simulink library "linkage_bushing_6DOF_lib"  (R2025a)
settings: Solver=VariableStepAuto  StartTime=0.0  StopTime=10.0  RelTol=1e-3
undefined symbols (not defined in the file): Connection, d_axialX, d_axialY, d_axialZ, d_torsX, d_torsY, d_torsZ, f_axialX_dam, f_axialX_spr, f_axialY_dam, f_axialY_spr, f_axialZ_dam, f_axialZ_spr, hp_joint, k_axialX, k_axialY, k_axialZ, k_torsX, k_torsY, k_torsZ, Linear, m_spr, m_sprX, m_sprZ, m_torsY, m_torsZ, m_torX, q_spr, q_sprX, q_sprZ, rhs_y, Table, v_axialX, v_axialY, v_axialZ, Visual, w_torsY, w_torsZ, w_torX, X, x_axialX, x_axialY, x_axialZ, Y, Z
libraries: sm_lib x22, Suspension_Utilities x7, $bdroot x3, bushing_forces_lib x2, linkage_bushing_5DOF_lib x1
(part 1 of 2)
Description:
  | Component of Simscape Vehicle Templates Library
  | 
  | Copyright 2018-2026 The MathWorks, Inc.
settings Model: Creator=smiller  LastModifiedBy=smiller
settings OptimizationCC: ReuseModelBlockBuffer=off
settings ModelReferenceCC: EnableRefExpFcnMdlSchedulingChecks=on
settings RTWCC: GPUComputeCapability=3.5

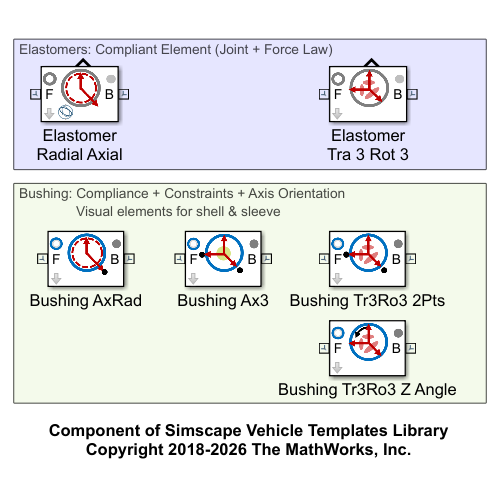
[thumbnail: Simulink's stored preview of the top-level diagram]
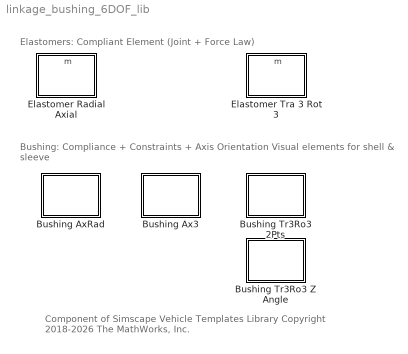
== system linkage_bushing_6DOF_lib ==
  note: Component of Simscape Vehicle Templates Library
      | Copyright 2018-2026 The MathWorks, Inc.
  note: Elastomers: Compliant Element (Joint + Force Law)
  note: Bushing: Compliance + Constraints + Axis Orientation
      |                Visual elements for shell & sleeve
  Bushing Ax3 : Subsystem  VariantControl=Bushing_Ax3  mask(Bushing with Independent Axial Compliance on 3-Axes (6-DOF)){checkbox_setTargets=on, leftOrRight=rhs_y, hp_j=hp_joint, hp_z=Connection.sAxialOrientationZ.Value, hp_x=Connection.sAxialOrientationX.Value, AxisAttachment=Connection.AxisAttachment.class.Value, sprx=Connection.SpringX, spry=Connection.SpringY, sprz=Connection.SpringZ, damx=Connection.DamperX, damy=Connection.DamperY, damz=Connection.DamperZ, shell_or=Visual.hp.rad*2, shell_len=Visual.hp.rad*2, shell_clr=Visual.BushingShell.clr, shell_opc=Visual.part.opc, sleeve_clr=Visual.Bushing.clr, sleeve_opc=Visual.part.opc}
      mask prompts: checkbox_setTargets "Set position targets to 0"; leftOrRight "Left (1) or Right (-1)"; hp_j "Joint HP [x  y z] (m)"; hp_z "Bushing Z-Axis Point [x y z] (m)"; hp_x "Bushing X-Axis Point [x y z] (m)"; AxisAttachment "Bushing Axes Attachment (string)"; sprx "Spring X Parameters (struct)"; spry "Spring Y Parameters (struct)"; sprz "Spring Z Parameters (struct)"; damx "Damper X Parameters (struct)"; damy "Damper Y Parameters (struct)"; damz "Damper Z Parameters (struct)"; shell_or "Shell Outer Radius (m)"; shell_len "Shell Length (m)"; shell_clr "Shell Color [R G B]"; shell_opc "Shell Opacity (0-1)"; sleeve_clr "Sleeve Color [R G B]"; sleeve_opc "Sleeve Opacity (0-1)"
      mask help: Models bushing compliance with independent force laws for x, y, and z directions. Select force laws that model compliance as linear or nonlinear.
      mask init:
      | curblk = gcb;
      | 
      | set_param([curblk '/Elastomer'],...
      |     'popup_force_law_spr_axiX', sprx.Law.Value,...
      |     'popup_force_law_spr_axiY', spry.Law.Value,...
      |     'popup_force_law_spr_axiZ', sprz.Law.Value,...
      |     'popup_force_law_dam_axiX', damx.Law.Value,...
      |     'popup_force_law_dam_axiY', damy.Law.Value,...
      |     'popup_force_law_dam_axiZ', damz.Law.Value...
      |     );
      | 
      | if(strcmp(AxisAttachment,'Inner'))
      |    set_param([curblk '/Inner'],'LabelModeActiveChoice','Fixed');
      |    set_param([curblk '/Outer'],'LabelModeActiveChoice','Gimbal');
      | elseif(strcmp(AxisAttachment,'Outer'))
      |    set_param([curblk '/Inner'],'LabelModeActiveChoice','Revolute');
      |    set_param([curblk '/Outer'],'LabelModeActiveChoice','Universal');
      | end
      | 
      | leftOrRight_vec = [1 leftOrRight 1];
      mask TypeOptions checkbox_setTargets: Inner/checkbox_setTargets | Outer/checkbox_setTargets | Elastomer/checkbox_setTargets
      mask TypeOptions hp_j: Elastomer/hp_j
      mask DialogControl cont_vis Prompt: Visualization
      mask Display: image('sm_car_bushing_tr3_perpaxial.png');
  Bushing AxRad : Subsystem  VariantControl=Bushing_AxRad  mask(Bushing with Radial and Axial Compliance, 6 DOF){checkbox_setTargets=on, leftOrRight=rhs_y, hp_j=hp_joint, hp_z=Connection.sAxialOrientationZ.Value, sprRad=Connection.RadialSpring, damRad=Connection.RadialDamper, sprAxi=Connection.AxialSpring, damAxi=Connection.AxialSpring, shell_or=Visual.hp.rad*2, shell_len=Visual.hp.rad*2, shell_clr=Visual.BushingShell.clr, shell_opc=Visual.part.opc, sleeve_clr=Visual.Bushing.clr, sleeve_opc=Visual.part.opc}
      mask prompts: checkbox_setTargets "Set position targets to 0"; leftOrRight "Left (1) or Right (-1)"; hp_j "Joint HP [x  y z] (m)"; hp_z "Bushing Z-Axis Point [x y z] (m)"; sprRad "Radial Spring Parameters (struct)"; damRad "Radial Darmper Parameters (struct)"; sprAxi "Axial Spring Parameters (struct)"; damAxi "Axial Damper Parameters (struct)"; shell_or "Shell Outer Radius (m)"; shell_len "Shell Length (m)"; shell_clr "Shell Color [R G B]"; shell_opc "Shell Opacity (0-1)"; sleeve_clr "Sleeve Color [R G B]"; sleeve_opc "Sleeve Opacity (0-1)"
      mask help: Models compliance with independent radial and axial force laws. Specify orientation of axial axis by defining the location of the bushing and the location of a point along that axis.
      mask init:
      | curblk = gcb;
      | set_param([curblk '/Elastomer'],...
      |     'popup_force_law_dam_rad', damRad.Law.Value,...
      |     'popup_force_law_spr_axi', sprAxi.Law.Value,...
      |     'popup_force_law_dam_axi', damAxi.Law.Value...
      |     );
      | set_param([curblk '/Elastomer'],...
      |     'popup_force_law_spr_rad', sprAxi.Law.Value);
      | 
      | leftOrRight_vec = [1 leftOrRight 1];
      mask TypeOptions checkbox_setTargets: Elastomer/checkbox_setTargets
      mask TypeOptions hp_j: Elastomer/hp_j
      mask DialogControl cont_vis Prompt: Visualization
      mask Display: image('sm_car_bushing_axrad_6dof.png');
  Bushing Tr3Ro3 2Pts : Subsystem  VariantControl=Bushing_Tr3Ro3  mask(Bushing with Axial and Torsional Compliance, Orient Two Points){checkbox_setTargets=on, leftOrRight=rhs_y, hp_j=hp_joint, hp_z=Connection.sAxialOrientationZ.Value, hp_x=Connection.sAxialOrientationX.Value, sprx=Connection.SpringX, spry=Connection.SpringY, sprz=Connection.SpringZ, damx=Connection.DamperX, damy=Connection.DamperY, damz=Connection.DamperZ, sprqx=Connection.SpringqX, sprqy=Connection.SpringqY, sprqz=Connection.SpringqZ, damqx=Connection.DamperqX, damqy=Connection.DamperqY, damqz=Connection.DamperqZ, shell_or=Visual.hp.rad*2, shell_len=Visual.hp.rad*2, shell_clr=Visual.BushingShell.clr, shell_opc=Visual.part.opc, sleeve_clr=Visual.Bushing.clr, sleeve_opc=Visual.part.opc}
      mask prompts: checkbox_setTargets "Set position targets to 0"; leftOrRight "Left (1) or Right (-1)"; hp_j "HP Joint [xyz] (m)"; hp_z "Bushing Z-Axis Point [x y z] (m)"; hp_x "Bushing X-Axis Point [x y z] (m)"; sprx "Spring X Parameters (struct)"; spry "Spring Y Parameters (struct)"; sprz "Spring Z Parameters (struct)"; damx "Damper X Parameters (struct)"; damy "Damper Y Parameters (struct)"; damz "Damper Z Parameters (struct)"; sprqx "Spring X Parameters (struct)"; sprqy "Spring Y Parameters (struct)"; sprqz "Spring Z Parameters (struct)"; damqx "Damper X Parameters (struct)"; damqy "Damper Y Parameters (struct)"; damqz "Damper Z Parameters (struct)"; shell_or "Shell Outer Radius (m)"; shell_len "Shell Length (m)"; shell_clr "Shell Color [R G B]"; shell_opc "Shell Opacity (0-1)"; sleeve_clr "Sleeve Color [R G B]"; sleeve_opc "Sleeve Opacity (0-1)"
      mask help: Models bushing compliance with independent force laws for translational and rotational stiffness and damping. The forces are parameterized along/about each local axis. Select force laws that model compliance as a linear coefficient or a lookup table. Orientation of z- and x- axes are defined by two points in 3D space.
      mask init:
      | curblk = gcb;
      | 
      | set_param([curblk '/Elastomer'],...
      |     'popup_force_law_spr_axiX', sprx.Law.Value,...
      |     'popup_force_law_spr_axiY', spry.Law.Value,...
      |     'popup_force_law_spr_axiZ', sprz.Law.Value,...
      |     'popup_force_law_dam_axiX', damx.Law.Value,...
      |     'popup_force_law_dam_axiY', damy.Law.Value,...
      |     'popup_force_law_dam_axiZ', damz.Law.Value,...
      |     'popup_force_law_spr_torX', sprqx.Law.Value,...
      |     'popup_force_law_spr_torY', sprqy.Law.Value,...
      |     'popup_force_law_spr_torZ', sprqz.Law.Value,...
      |     'popup_force_law_dam_torX', damqx.Law.Value,...
      |     'popup_force_law_dam_torY', damqy.Law.Value,...
      |     'popup_force_law_dam_torZ', damqz.Law.Value...
      |     );
      | 
      | leftOrRight_vec = [1 leftOrRight 1];
      mask TypeOptions checkbox_setTargets: Elastomer/checkbox_setTargets
      mask DialogControl cont_trans Prompt: Translational
      mask DialogControl cont_rot Prompt: Rotational
      mask DialogControl cont_vis Prompt: Visualization
      mask Display: image('sm_car_bushing_tr3ro3_2pts.png');
  Bushing Tr3Ro3 Z Angle : Subsystem  VariantControl=Bushing_Tr3Ro3  mask(Bushing with Axial and Torsional Compliance, Orient Z-Axis Rotation){checkbox_setTargets=on, leftOrRight=rhs_y, qOriZ=Connection.qOriZ.Value, sprx=Connection.SpringX, spry=Connection.SpringY, sprz=Connection.SpringZ, damx=Connection.DamperX, damy=Connection.DamperY, damz=Connection.DamperZ, sprqx=Connection.SpringqX, sprqy=Connection.SpringqY, sprqz=Connection.SpringqZ, damqx=Connection.DamperqX, damqy=Connection.DamperqY, damqz=Connection.DamperqZ, shell_or=Visual.hp.rad*2, shell_len=Visual.hp.rad*2, shell_clr=Visual.BushingShell.clr, shell_opc=Visual.part.opc, sleeve_clr=Visual.Bushing.clr, sleeve_opc=Visual.part.opc}
      mask prompts: checkbox_setTargets "Set position targets to 0"; leftOrRight "Left (1) or Right (-1)"; qOriZ "Z-Axis Rotation (deg)"; sprx "Spring X Parameters (struct)"; spry "Spring Y Parameters (struct)"; sprz "Spring Z Parameters (struct)"; damx "Damper X Parameters (struct)"; damy "Damper Y Parameters (struct)"; damz "Damper Z Parameters (struct)"; sprqx "Spring X Parameters (struct)"; sprqy "Spring Y Parameters (struct)"; sprqz "Spring Z Parameters (struct)"; damqx "Damper X Parameters (struct)"; damqy "Damper Y Parameters (struct)"; damqz "Damper Z Parameters (struct)"; shell_or "Shell Outer Radius (m)"; shell_len "Shell Length (m)"; shell_clr "Shell Color [R G B]"; shell_opc "Shell Opacity (0-1)"; sleeve_clr "Sleeve Color [R G B]"; sleeve_opc "Sleeve Opacity (0-1)"
      mask help: Models bushing compliance with independent force laws for translational and rotational stiffness and damping. The forces are parameterized along/about each local axis. Select force laws that model compliance as a linear coefficient or a lookup table. Orientation of x- and y-axis are defined a rotation angle about the z-axis.
      mask init: same as linkage_bushing_6DOF_lib/Bushing Tr3Ro3 2Pts
      mask TypeOptions checkbox_setTargets: Elastomer/checkbox_setTargets
      mask DialogControl cont_trans Prompt: Translational
      mask DialogControl cont_rot Prompt: Rotational
      mask DialogControl cont_vis Prompt: Visualization
      mask Display: image('sm_car_bushing_tr3ro3_zangle.png')
  Elastomer Radial Axial : Subsystem  mask(Elastomer with Radial and Axial Compliance (6-DOF)){checkbox_setTargets=off, popup_force_law_spr_rad=Linear, k_radial=20, x_radial=[-4, -3, -2, -1, 0, 1, 2, 3, 4], f_radial_spr=[-4, -3, -2, -1, 0, 1, 2, 3, 4]*10, k1_radial_max=3.0139e+03, b1_radial_max=11471, x_radial_max=[-3 -1.5 1.5 3]*1e-3, f_radial_max=[-10 -4 4 10]*655.5098, popup_force_law_dam_rad=Linear, d_radial=20, v_radial=[-4, -3, -2, -1, 0, 1, 2, 3, 4], f_radial_dam=[-4, -3, -2, -1, 0, 1, 2, 3, 4]*10, popup_force_law_spr_axi=Linear, k_axial=20, x_axial=[-4, -3, -2, -1, 0, 1, 2, 3, 4], f_axial_spr=[-4, -3, -2, -1, 0, 1, 2, 3, 4]*10, popup_force_law_dam_axi=Linear, d_axial=20, v_axial=[-4, -3, -2, -1, 0, 1, 2, 3, 4], f_axial_dam=[-4, -3, -2, -1, 0, 1, 2, 3, 4]*10, shell_or=Visual.hp.rad*2, elastomer_ir=Visual.hp.rad, shell_len=Visual.hp.rad*4, elastomer_clr=Visual.Bushing.clr, elastomer_opc=Visual.part.opc}
      mask prompts: checkbox_setTargets "Set position targets to 0"; popup_force_law_spr_rad "Spring Force Law"; k_radial "Spring Coefficient (N/mm)"; x_radial "Spring Deflection [min max] (mm)"; f_radial_spr "Spring Force [min max] (N)"; k1_radial_max "Maxwell k1"; b1_radial_max "Maxwell b1"; x_radial_max "Maxwell Displacement [min max] (mm)"; f_radial_max "Maxwell Force [min max] (N)"; popup_force_law_dam_rad "Damper Force Law"; d_radial "Damper Coefficient (N/(m/s))"; v_radial "Damper Velocity [min max] (m/s)"; f_radial_dam "Damper Force [min max] (N)"; popup_force_law_spr_axi "Spring Force Law"; k_axial "Spring Coefficient (N/mm)"; x_axial "Spring Displacement [min max] (mm)"; f_axial_spr "Spring Force [min max] (N)"; popup_force_law_dam_axi "Damper Force Law"; d_axial "Damper Coefficient (N/(m/s))"; v_axial "Damper Velocity [min max] (m/s)"; f_axial_dam "Damper Force [min max] (N)"; shell_or "Shell Outer Radius (m)"; elastomer_ir "Elastomer Inner Radius (m)"; shell_len "Shell Length (m)"; elastomer_clr "Elastomer Color [R G B]"; elastomer_opc "Elastomer Opacity [R G B]"
      mask help: Models elastomer compliance with independent force laws for radial (x-y plane) and axial (z-axis) directions. Select force laws that model compliance as linear, nonlinear, or nonlinear with hysteresis. All 6 degrees of freedom are provided within this block to make the overall model more efficient.
      mask init:
      | curblk = gcb;
      | if(checkbox_setTargets)
      |     set_param([curblk '/Elastomer Joint'],...
      |         'PxPositionTargetSpecify','on',...
      |         'PyPositionTargetSpecify','on',...
      |         'PzPositionTargetSpecify','on',...
      |         'RxPositionTargetSpecify','on',...
      |         'RyPositionTargetSpecify','on',...
      |         'RzPositionTargetSpecify','on'...
      |         );
      | else
      |     set_param([curblk '/Elastomer Joint'],...
      |         'PxPositionTargetSpecify','off',...
      |         'PyPositionTargetSpecify','off',...
      |         'PzPositionTargetSpecify','off',...
      |         'RxPositionTargetSpecify','off',...
      |         'RyPositionTargetSpecify','off',...
      |         'RzPositionTargetSpecify','off'...
      |         );
      | end
      settings: PortSchema="{\"entries\":[{\"content\":{\"sides\":[{\"content\":{\"connectorIds\":[\"LConn1\"]},\"type\":\"ConnectorPlacement.EquallySpacedRectSide\",\"uuid\":\"540bb151-3239-4a9d-82ba-b7afa97281a8\"},{\"content\":{\"connectorIds\":[\"RConn1\"],\"side\":\"RIGHT\"},\"type\":\"ConnectorPlacement.EquallySpacedRectSide\",\"uuid\":\"0af2999e-e304-4113-9c38-08ac5dd2068d\"},{\"content\":{\"connectorIds\":[\"Out1\"],\"side\":\"TOP\"},\"type\":\"ConnectorPlacement.EquallySpacedRectSide\",\"uuid\":\"c7e19545-6bd3-4656-b994-719fb436eca6\"}]},\"type\":\"ConnectorPlacement.EquallySpacedConnector\",\"uuid\":\"c532a1d4-44be-42d7-8101-c903e69d0a9b\"}],\"packageUris\":[\"http://schema.mathworks.com/mf0/Connector/R2020b\"],\"version\":\"1.0\"}"
      mask TypeOptions popup_force_law_spr_rad: Force Law/popup_force_law_spr_rad
      mask Callback popup_force_law_spr_rad:
      | maskObj = Simulink.Mask.get(gcb); % Get the mask object of the current block
      | krad_h  = maskObj.getParameter('k_radial'); % Get the parameter to hide
      | 
      | xrad_h  = maskObj.getParameter('x_radial'); % Get the parameter to hide
      | fSrad_h = maskObj.getParameter('f_radial_spr'); % Get the parameter to hide
      | k1rad_h  = maskObj.getParameter('k1_radial_max'); % Get the parameter to hide
      | b1rad_h  = maskObj.getParameter('b1_radial_max'); % Get the parameter to hide
      | xmrad_h  = maskObj.getParameter('x_radial_max'); % Get the parameter to hide
      | fmrad_h  = maskObj.getParameter('f_radial_max'); % Get the parameter to hide
      | 
      | % Check the value of ControlParam
      | frcLawSpr = get_param(gcb, 'popup_force_law_spr_rad');
      | 
      | krad_h.Visible  = 'off';
      | xrad_h.Visible  = 'off';
      | fSrad_h.Visible = 'off';
      | k1rad_h.Visible  = 'off';
      | b1rad_h.Visible  = 'off';
      | xmrad_h.Visible  = 'off';
      | fmrad_h.Visible  = 'off';
      | 
      | if strcmp(frcLawSpr, 'Linear')
      |     krad_h.Visible  = 'on';
      | elseif strcmp(frcLawSpr, 'Table')
      |     xrad_h.Visible  = 'on';
      |     fSrad_h.Visible = 'on';
      | elseif strcmp(frcLawSpr, 'Maxwell_SLS')
      |     k1rad_h.Visible  = 'on';
      |     b1rad_h.Visible = 'on';
      |     xmrad_h.Visible = 'on';
      |     fmrad_h.Visible = 'on';
      | end
      mask TypeOptions k_radial: Force Law/k_radial
      mask TypeOptions x_radial: Force Law/x_radial
      mask TypeOptions f_radial_spr: Force Law/f_radial_spr
      mask TypeOptions k1_radial_max: Force Law/k1_radial_max
      mask TypeOptions b1_radial_max: Force Law/b1_radial_max
      mask TypeOptions x_radial_max: Force Law/x_radial_max
      mask TypeOptions f_radial_max: Force Law/f_radial_max
      mask TypeOptions popup_force_law_dam_rad: Force Law/popup_force_law_dam_rad
      mask Callback popup_force_law_dam_rad:
      | maskObj = Simulink.Mask.get(gcb); % Get the mask object of the current block
      | drad_h  = maskObj.getParameter('d_radial'); % Get the parameter to hide
      | 
      | vrad_h  = maskObj.getParameter('v_radial'); % Get the parameter to hide
      | fDrad_h = maskObj.getParameter('f_radial_dam'); % Get the parameter to hide
      | 
      | % Check the value of ControlParam
      | frcLawDam = get_param(gcb, 'popup_force_law_dam_rad');
      | 
      | drad_h.Visible  = 'off';
      | vrad_h.Visible  = 'off';
      | fDrad_h.Visible = 'off';
      | 
      | if strcmp(frcLawDam, 'Linear')
      |     drad_h.Visible  = 'on';
      | elseif strcmp(frcLawDam, 'Table')
      |     vrad_h.Visible  = 'on';
      |     fDrad_h.Visible = 'on';
      | end
      mask TypeOptions d_radial: Force Law/d_radial
      mask TypeOptions v_radial: Force Law/v_radial
      mask TypeOptions f_radial_dam: Force Law/f_radial_dam
      mask TypeOptions popup_force_law_spr_axi: Force Law/popup_force_law_spr_axi
      mask Callback popup_force_law_spr_axi:
      | maskObj = Simulink.Mask.get(gcb); % Get the mask object of the current block
      | kaxi_h  = maskObj.getParameter('k_axial'); % Get the parameter to hide
      | 
      | xaxi_h  = maskObj.getParameter('x_axial'); % Get the parameter to hide
      | fSaxi_h  = maskObj.getParameter('f_axial_spr'); % Get the parameter to hide
      | 
      | % Check the value of ControlParam
      | controlParamValue = get_param(gcb, 'popup_force_law_spr_axi');
      | 
      | kaxi_h.Visible  = 'off';
      | xaxi_h.Visible  = 'off';
      | fSaxi_h.Visible  = 'off';
      | 
      | if strcmp(controlParamValue, 'Linear')
      |     kaxi_h.Visible  = 'on';
      | else
      |     xaxi_h.Visible  = 'on';
      |     fSaxi_h.Visible  = 'on';
      | end
      mask TypeOptions k_axial: Force Law/k_axial
      mask TypeOptions x_axial: Force Law/x_axial
      mask TypeOptions f_axial_spr: Force Law/f_axial_spr
      mask TypeOptions popup_force_law_dam_axi: Force Law/popup_force_law_dam_axi
      mask Callback popup_force_law_dam_axi:
      | maskObj = Simulink.Mask.get(gcb); % Get the mask object of the current block
      | daxi_h  = maskObj.getParameter('d_axial'); % Get the parameter to hide
      | 
      | vaxi_h  = maskObj.getParameter('v_axial'); % Get the parameter to hide
      | fDaxi_h  = maskObj.getParameter('f_axial_dam'); % Get the parameter to hide
      | 
      | % Check the value of ControlParam
      | controlParamValue = get_param(gcb, 'popup_force_law_dam_axi');
      | 
      | daxi_h.Visible  = 'off';
      | vaxi_h.Visible  = 'off';
      | fDaxi_h.Visible  = 'off';
      | 
      | if strcmp(controlParamValue, 'Linear')
      |     daxi_h.Visible  = 'on';
      | else
      |     vaxi_h.Visible  = 'on';
      |     fDaxi_h.Visible  = 'on';
      | end
      mask TypeOptions d_axial: Force Law/d_axial
      mask TypeOptions v_axial: Force Law/v_axial
      mask TypeOptions f_axial_dam: Force Law/f_axial_dam
      mask DialogControl cont_radial Prompt: Radial
      mask DialogControl cont_axial Prompt: Axial
      mask DialogControl cont_vis Prompt: Visualization
      mask Display: image('sm_car_elastomer_axrad_6dof.png');
  Elastomer Tra 3 Rot 3 : Subsystem  mask(Elastomer with Axial  and Torsional Compliance){checkbox_setTargets=off, popup_force_law_spr_axiX=Table, k_axialX=k_axialX, x_axialX=x_axialX, f_axialX_spr=f_axialX_spr, popup_force_law_dam_axiX=Linear, d_axialX=d_axialX, v_axialX=v_axialX, f_axialX_dam=f_axialX_dam, popup_force_law_spr_axiY=Linear, k_axialY=k_axialY, x_axialY=x_axialY, f_axialY_spr=f_axialY_spr, popup_force_law_dam_axiY=Linear, d_axialY=d_axialY, v_axialY=v_axialY, f_axialY_dam=f_axialY_dam, popup_force_law_spr_axiZ=Linear, k_axialZ=k_axialZ, x_axialZ=x_axialZ, f_axialZ_spr=f_axialZ_spr, popup_force_law_dam_axiZ=Linear, d_axialZ=d_axialZ, v_axialZ=v_axialZ, f_axialZ_dam=f_axialZ_dam, popup_force_law_spr_torX=Linear, k_torsX=k_torsX, q_sprX=q_sprX, m_sprX=m_sprX, popup_force_law_dam_torX=Linear, d_torsX=d_torsX, w_torsX=w_torX, m_torsX=m_torX, popup_force_law_spr_torY=Table, k_torsY=k_torsY, q_sprY=q_spr, m_sprY=m_spr, popup_force_law_dam_torY=Table, d_torsY=d_torsY, w_torsY=w_torsY, m_torsY=m_torsY, popup_force_law_spr_torZ=Linear, k_torsZ=k_torsZ, q_sprZ=q_sprZ, m_sprZ=m_sprZ, popup_force_law_dam_torZ=Linear, d_torsZ=d_torsZ, w_torsZ=w_torsZ, m_torsZ=m_torsZ, shell_or=Visual.hp.rad*2, elastomer_ir=Visual.hp.rad, shell_len=Visual.hp.rad*2, elastomer_clr=Visual.Bushing.clr, elastomer_opc=Visual.part.opc, elastomer_axis_clr=Visual.BushingXAxis.clr}
      mask prompts: checkbox_setTargets "Set position targets to 0"; popup_force_law_spr_axiX "Spring Force Law"; k_axialX "Spring Coefficient (N/mm)"; x_axialX "Spring Displacement [min max] (mm)"; f_axialX_spr "Spring Force [min max] (N)"; popup_force_law_dam_axiX "Damper Force Law"; d_axialX "Damper Coefficient (N/(m/s))"; v_axialX "Damper Velocity [min max] (m/s)"; f_axialX_dam "Damper Force [min max] (N)"; popup_force_law_spr_axiY "Spring Force Law"; k_axialY "Spring Coefficient (N/mm)"; x_axialY "Spring Displacement [min max] (mm)"; f_axialY_spr "Spring Force [min max] (N)"; popup_force_law_dam_axiY "Damper Force Law"; d_axialY "Damper Coefficient (N/(m/s))"; v_axialY "Damper Velocity [min max] (m/s)"; f_axialY_dam "Damper Force [min max] (N)"; popup_force_law_spr_axiZ "Spring Force Law"; k_axialZ "Spring Coefficient (N/mm)"; x_axialZ "Spring Displacement [min max] (mm)"; f_axialZ_spr "Spring Force [min max] (N)"; popup_force_law_dam_axiZ "Damper Force Law"; d_axialZ "Damper Coefficient (N/(m/s))"; v_axialZ "Damper Velocity [min max] (m/s)"; f_axialZ_dam "Damper Force [min max] (N)"; popup_force_law_spr_torX "Spring Force Law"; k_torsX "Spring Coefficient  (N*m/deg)"; q_sprX "Spring Displacement [min max] (deg)"; m_sprX "Spring Torque [min max] (N*m)"; popup_force_law_dam_torX "Damper Force Law"; d_torsX "Damper Coefficient (N*m/(deg/s))"; w_torsX "Damper Velocity [min max] (deg/s)"; m_torsX "Damper Torque [min max] (N*m)"; popup_force_law_spr_torY "Spring Force Law"; k_torsY "Spring Coefficient (N*m/deg)"; q_sprY "Spring Displacement [min max] (deg)"; m_sprY "Spring Torque [min max] (N*m)"; popup_force_law_dam_torY "Damper Force Law"; d_torsY "Damper Coefficient (N*m/(deg/s))"; w_torsY "Damper Velocity [min max] (deg/s)"; m_torsY "Damper Torque [min max] (N*m)"; popup_force_law_spr_torZ "Spring Force Law"; k_torsZ "Spring Coefficient (N*m/deg)"; q_sprZ "Spring Displacement [min max] (deg)"; m_sprZ "Spring Torque [min max] (N*m)"; popup_force_law_dam_torZ "Damper Force Law"; d_torsZ "Damper Coefficient (N*m/(deg/s))"; w_torsZ "Damper Velocity [min max] (deg/s)"; m_torsZ "Damper Torque [min max] (N*m)"; shell_or "Shell Outer Radius (m)"; elastomer_ir "Elastomer Inner Radius (m)"; shell_len "Shell Length (m)"; elastomer_clr "Elastomer Color [R G B]"; elastomer_opc "Elastomer Opacity [R G B]"; elastomer_axis_clr "Elastomer Axis Color [R G B]"
      mask help: Models elastomer compliance with independent force laws for translational and rotational stiffness and damping. The forces are parameterized along/about each local axis. Select force laws that model compliance as a linear coefficient or a lookup table.
      mask init: same as linkage_bushing_6DOF_lib/Elastomer Radial Axial
      settings: PortSchema="{\"entries\":[{\"content\":{\"sides\":[{\"content\":{\"connectorIds\":[\"LConn1\"]},\"type\":\"ConnectorPlacement.EquallySpacedRectSide\",\"uuid\":\"540bb151-3239-4a9d-82ba-b7afa97281a8\"},{\"content\":{\"connectorIds\":[\"RConn1\"],\"side\":\"RIGHT\"},\"type\":\"ConnectorPlacement.EquallySpacedRectSide\",\"uuid\":\"0af2999e-e304-4113-9c38-08ac5dd2068d\"},{\"content\":{\"connectorIds\":[\"Out1\"],\"side\":\"TOP\"},\"type\":\"ConnectorPlacement.EquallySpacedRectSide\",\"uuid\":\"c7e19545-6bd3-4656-b994-719fb436eca6\"}]},\"type\":\"ConnectorPlacement.EquallySpacedConnector\",\"uuid\":\"c532a1d4-44be-42d7-8101-c903e69d0a9b\"}],\"packageUris\":[\"http://schema.mathworks.com/mf0/Connector/R2020b\"],\"version\":\"1.0\"}"
      mask TypeOptions popup_force_law_spr_axiX: Force Law/popup_force_law_spr_axiX
      mask Callback popup_force_law_spr_axiX:
      | maskObj = Simulink.Mask.get(gcb); % Get the mask object of the current block
      | kaxiX_h  = maskObj.getParameter('k_axialX'); % Get the parameter to hide
      | 
      | xaxiX_h  = maskObj.getParameter('x_axialX'); % Get the parameter to hide
      | fSaxiX_h  = maskObj.getParameter('f_axialX_spr'); % Get the parameter to hide
      | 
      | % Check the value of ControlParam
      | controlParamValue = get_param(gcb, 'popup_force_law_spr_axiX');
      | 
      | kaxiX_h.Visible  = 'off';
      | xaxiX_h.Visible  = 'off';
      | fSaxiX_h.Visible  = 'off';
      | 
      | if strcmp(controlParamValue, 'Linear')
      |     kaxiX_h.Visible  = 'on';
      | else
      |     xaxiX_h.Visible  = 'on';
      |     fSaxiX_h.Visible  = 'on';
      | end
      mask TypeOptions k_axialX: Force Law/k_axialX
      mask TypeOptions x_axialX: Force Law/x_axialX
      mask TypeOptions f_axialX_spr: Force Law/f_axialX_spr
      mask TypeOptions popup_force_law_dam_axiX: Force Law/popup_force_law_dam_axiX
      mask Callback popup_force_law_dam_axiX:
      | maskObj = Simulink.Mask.get(gcb); % Get the mask object of the current block
      | daxiX_h  = maskObj.getParameter('d_axialX'); % Get the parameter to hide
      | 
      | vaxiX_h  = maskObj.getParameter('v_axialX'); % Get the parameter to hide
      | fDaxiX_h  = maskObj.getParameter('f_axialX_dam'); % Get the parameter to hide
      | 
      | % Check the value of ControlParam
      | controlParamValue = get_param(gcb, 'popup_force_law_dam_axiX');
      | 
      | daxiX_h.Visible  = 'off';
      | vaxiX_h.Visible  = 'off';
      | fDaxiX_h.Visible  = 'off';
      | 
      | if strcmp(controlParamValue, 'Linear')
      |     daxiX_h.Visible  = 'on';
      | else
      |     vaxiX_h.Visible  = 'on';
      |     fDaxiX_h.Visible  = 'on';
      | end
      mask TypeOptions d_axialX: Force Law/d_axialX
      mask TypeOptions v_axialX: Force Law/v_axialX
      mask TypeOptions f_axialX_dam: Force Law/f_axialX_dam
      mask TypeOptions popup_force_law_spr_axiY: Force Law/popup_force_law_spr_axiY
      mask Callback popup_force_law_spr_axiY:
      | maskObj = Simulink.Mask.get(gcb); % Get the mask object of the current block
      | kaxiY_h  = maskObj.getParameter('k_axialY'); % Get the parameter to hide
      | 
      | xaxiY_h  = maskObj.getParameter('x_axialY'); % Get the parameter to hide
      | fSaxiY_h  = maskObj.getParameter('f_axialY_spr'); % Get the parameter to hide
      | 
      | % Check the value of ControlParam
      | controlParamValue = get_param(gcb, 'popup_force_law_spr_axiY');
      | 
      | kaxiY_h.Visible  = 'off';
      | xaxiY_h.Visible  = 'off';
      | fSaxiY_h.Visible  = 'off';
      | 
      | if strcmp(controlParamValue, 'Linear')
      |     kaxiY_h.Visible  = 'on';
      | else
      |     xaxiY_h.Visible  = 'on';
      |     fSaxiY_h.Visible  = 'on';
      | end
      mask TypeOptions k_axialY: Force Law/k_axialY
      mask TypeOptions x_axialY: Force Law/x_axialY
      mask TypeOptions f_axialY_spr: Force Law/f_axialY_spr
      mask TypeOptions popup_force_law_dam_axiY: Force Law/popup_force_law_dam_axiY
      mask Callback popup_force_law_dam_axiY:
      | maskObj = Simulink.Mask.get(gcb); % Get the mask object of the current block
      | daxiY_h  = maskObj.getParameter('d_axialY'); % Get the parameter to hide
      | 
      | vaxiY_h  = maskObj.getParameter('v_axialY'); % Get the parameter to hide
      | fDaxiY_h  = maskObj.getParameter('f_axialY_dam'); % Get the parameter to hide
      | 
      | % Check the value of ControlParam
      | controlParamValue = get_param(gcb, 'popup_force_law_dam_axiY');
      | 
      | daxiY_h.Visible  = 'off';
      | vaxiY_h.Visible  = 'off';
      | fDaxiY_h.Visible  = 'off';
      | 
      | if strcmp(controlParamValue, 'Linear')
      |     daxiY_h.Visible  = 'on';
      | else
      |     vaxiY_h.Visible  = 'on';
      |     fDaxiY_h.Visible  = 'on';
      | end
      mask TypeOptions d_axialY: Force Law/d_axialY
      mask TypeOptions v_axialY: Force Law/v_axialY
      mask TypeOptions f_axialY_dam: Force Law/f_axialY_dam
      mask TypeOptions popup_force_law_spr_axiZ: Force Law/popup_force_law_spr_axiZ
      mask Callback popup_force_law_spr_axiZ:
      | maskObj = Simulink.Mask.get(gcb); % Get the mask object of the current block
      | kaxiZ_h  = maskObj.getParameter('k_axialZ'); % Get the parameter to hide
      | 
      | xaxiZ_h  = maskObj.getParameter('x_axialZ'); % Get the parameter to hide
      | fSaxiZ_h  = maskObj.getParameter('f_axialZ_spr'); % Get the parameter to hide
      | 
      | % Check the value of ControlParam
      | controlParamValue = get_param(gcb, 'popup_force_law_spr_axiZ');
      | 
      | kaxiZ_h.Visible  = 'off';
      | xaxiZ_h.Visible  = 'off';
      | fSaxiZ_h.Visible  = 'off';
      | 
      | if strcmp(controlParamValue, 'Linear')
      |     kaxiZ_h.Visible  = 'on';
      | else
      |     xaxiZ_h.Visible  = 'on';
      |     fSaxiZ_h.Visible  = 'on';
      | end
      mask TypeOptions k_axialZ: Force Law/k_axialZ
      mask TypeOptions x_axialZ: Force Law/x_axialZ
      mask TypeOptions f_axialZ_spr: Force Law/f_axialZ_spr
      mask TypeOptions popup_force_law_dam_axiZ: Force Law/popup_force_law_dam_axiZ
      mask Callback popup_force_law_dam_axiZ:
      | maskObj = Simulink.Mask.get(gcb); % Get the mask object of the current block
      | daxiZ_h  = maskObj.getParameter('d_axialZ'); % Get the parameter to hide
      | 
      | vaxiZ_h  = maskObj.getParameter('v_axialZ'); % Get the parameter to hide
      | fDaxiZ_h  = maskObj.getParameter('f_axialZ_dam'); % Get the parameter to hide
      | 
      | % Check the value of ControlParam
      | controlParamValue = get_param(gcb, 'popup_force_law_dam_axiZ');
      | 
      | daxiZ_h.Visible  = 'off';
      | vaxiZ_h.Visible  = 'off';
      | fDaxiZ_h.Visible  = 'off';
      | 
      | if strcmp(controlParamValue, 'Linear')
      |     daxiZ_h.Visible  = 'on';
      | else
      |     vaxiZ_h.Visible  = 'on';
      |     fDaxiZ_h.Visible  = 'on';
      | end
      mask TypeOptions d_axialZ: Force Law/d_axialZ
      mask TypeOptions v_axialZ: Force Law/v_axialZ
      mask TypeOptions f_axialZ_dam: Force Law/f_axialZ_dam
      mask TypeOptions popup_force_law_spr_torX: Force Law/popup_force_law_spr_torX
      mask Callback popup_force_law_spr_torX:
      | maskObj = Simulink.Mask.get(gcb); % Get the mask object of the current block
      | ktorX_h  = maskObj.getParameter('k_torsX'); % Get the parameter to hide
      | 
      | qsprX_h  = maskObj.getParameter('q_sprX'); % Get the parameter to hide
      | msprX_h  = maskObj.getParameter('m_sprX'); % Get the parameter to hide
      | 
      | % Check the value of ControlParam
      | controlParamValue = get_param(gcb, 'popup_force_law_spr_torX');
      | 
      | ktorX_h.Visible  = 'off';
      | qsprX_h.Visible  = 'off';
      | msprX_h.Visible  = 'off';
      | 
      | if strcmp(controlParamValue, 'Linear')
      |     ktorX_h.Visible  = 'on';
      | elseif strcmp(controlParamValue, 'Table')
      |     qsprX_h.Visible  = 'on';
      |     msprX_h.Visible  = 'on';
      | end
      mask TypeOptions k_torsX: Force Law/k_torsX
      mask TypeOptions q_sprX: Force Law/q_sprX
      mask TypeOptions m_sprX: Force Law/m_sprX
      mask TypeOptions popup_force_law_dam_torX: Force Law/popup_force_law_dam_torX
      mask Callback popup_force_law_dam_torX:
      | maskObj = Simulink.Mask.get(gcb); % Get the mask object of the current block
      | dtorX_h  = maskObj.getParameter('d_torsX'); % Get the parameter to hide
      | 
      | wtorX_h  = maskObj.getParameter('w_torsX'); % Get the parameter to hide
      | mtorX_h  = maskObj.getParameter('m_torsX'); % Get the parameter to hide
      | 
      | % Check the value of ControlParam
      | controlParamValue = get_param(gcb, 'popup_force_law_dam_torX');
      | 
      | dtorX_h.Visible  = 'off';
      | wtorX_h.Visible  = 'off';
      | mtorX_h.Visible  = 'off';
      | 
      | if strcmp(controlParamValue, 'Linear')
      |     dtorX_h.Visible  = 'on';
      | else
      |     wtorX_h.Visible  = 'on';
      |     mtorX_h.Visible  = 'on';
      | end
      mask TypeOptions d_torsX: Force Law/d_torsX
      mask TypeOptions w_torsX: Force Law/w_torsX
      mask TypeOptions m_torsX: Force Law/m_torsX
      mask TypeOptions popup_force_law_spr_torY: Force Law/popup_force_law_spr_torY
      mask Callback popup_force_law_spr_torY:
      | maskObj = Simulink.Mask.get(gcb); % Get the mask object of the current block
      | ktorY_h  = maskObj.getParameter('k_torsY'); % Get the parameter to hide
      | 
      | qsprY_h  = maskObj.getParameter('q_sprY'); % Get the parameter to hide
      | msprY_h  = maskObj.getParameter('m_sprY'); % Get the parameter to hide
      | 
      | % Check the value of ControlParam
      | controlParamValue = get_param(gcb, 'popup_force_law_spr_torY');
      | 
      | ktorY_h.Visible  = 'off';
      | qsprY_h.Visible  = 'off';
      | msprY_h.Visible  = 'off';
      | 
      | if strcmp(controlParamValue, 'Linear')
      |     ktorY_h.Visible  = 'on';
      | elseif strcmp(controlParamValue, 'Table')
      |     qsprY_h.Visible  = 'on';
      |     msprY_h.Visible  = 'on';
      | end
      mask TypeOptions k_torsY: Force Law/k_torsY
      mask TypeOptions q_sprY: Force Law/q_sprY
      mask TypeOptions m_sprY: Force Law/m_sprY
      mask TypeOptions popup_force_law_dam_torY: Force Law/popup_force_law_dam_torY
      mask Callback popup_force_law_dam_torY:
      | maskObj = Simulink.Mask.get(gcb); % Get the mask object of the current block
      | dtorY_h  = maskObj.getParameter('d_torsY'); % Get the parameter to hide
      | 
      | wtorY_h  = maskObj.getParameter('w_torsY'); % Get the parameter to hide
      | mtorY_h  = maskObj.getParameter('m_torsY'); % Get the parameter to hide
      | 
      | % Check the value of ControlParam
      | controlParamValue = get_param(gcb, 'popup_force_law_dam_torY');
      | 
      | dtorY_h.Visible  = 'off';
      | wtorY_h.Visible  = 'off';
      | mtorY_h.Visible  = 'off';
      | 
      | if strcmp(controlParamValue, 'Linear')
      |     dtorY_h.Visible  = 'on';
      | else
      |     wtorY_h.Visible  = 'on';
      |     mtorY_h.Visible  = 'on';
      | end
      mask TypeOptions d_torsY: Force Law/d_torsY
      mask TypeOptions w_torsY: Force Law/w_torsY
      mask TypeOptions m_torsY: Force Law/m_torsY
      mask TypeOptions popup_force_law_spr_torZ: Force Law/popup_force_law_spr_torZ
      mask Callback popup_force_law_spr_torZ:
      | maskObj = Simulink.Mask.get(gcb); % Get the mask object of the current block
      | ktorZ_h  = maskObj.getParameter('k_torsZ'); % Get the parameter to hide
      | 
      | qsprZ_h  = maskObj.getParameter('q_sprZ'); % Get the parameter to hide
      | msprZ_h  = maskObj.getParameter('m_sprZ'); % Get the parameter to hide
      | 
      | % Check the value of ControlParam
      | controlParamValue = get_param(gcb, 'popup_force_law_spr_torZ');
      | 
      | ktorZ_h.Visible  = 'off';
      | qsprZ_h.Visible  = 'off';
      | msprZ_h.Visible  = 'off';
      | 
      | if strcmp(controlParamValue, 'Linear')
      |     ktorZ_h.Visible  = 'on';
      | elseif strcmp(controlParamValue, 'Table')
      |     qsprZ_h.Visible  = 'on';
      |     msprZ_h.Visible  = 'on';
      | end
      mask TypeOptions k_torsZ: Force Law/k_torsZ
      mask TypeOptions q_sprZ: Force Law/q_sprZ
      mask TypeOptions m_sprZ: Force Law/m_sprZ
      mask TypeOptions popup_force_law_dam_torZ: Force Law/popup_force_law_dam_torZ
      mask Callback popup_force_law_dam_torZ:
      | maskObj = Simulink.Mask.get(gcb); % Get the mask object of the current block
      | dtorZ_h  = maskObj.getParameter('d_torsZ'); % Get the parameter to hide
      | 
      | wtorZ_h  = maskObj.getParameter('w_torsZ'); % Get the parameter to hide
      | mtorZ_h  = maskObj.getParameter('m_torsZ'); % Get the parameter to hide
      | 
      | % Check the value of ControlParam
      | controlParamValue = get_param(gcb, 'popup_force_law_dam_torZ');
      | 
      | dtorZ_h.Visible  = 'off';
      | wtorZ_h.Visible  = 'off';
      | mtorZ_h.Visible  = 'off';
      | 
      | if strcmp(controlParamValue, 'Linear')
      |     dtorZ_h.Visible  = 'on';
      | else
      |     wtorZ_h.Visible  = 'on';
      |     mtorZ_h.Visible  = 'on';
      | end
      mask TypeOptions d_torsZ: Force Law/d_torsZ
      mask TypeOptions w_torsZ: Force Law/w_torsZ
      mask TypeOptions m_torsZ: Force Law/m_torsZ
      mask DialogControl cont_axialX Prompt: Axial (local x)
      mask DialogControl cont_axialY Prompt: Axial (local y)
      mask DialogControl cont_axialZ Prompt: Axial (local z)
      mask DialogControl cont_torsX Prompt: Torsional (local x)
      mask DialogControl cont_torsY Prompt: Torsional (local y)
      mask DialogControl cont_torsZ Prompt: Torsional (local z)
      mask DialogControl cont_vis Prompt: Visualization
      mask Display: image('sm_car_elastomer_tr3ro3.png');

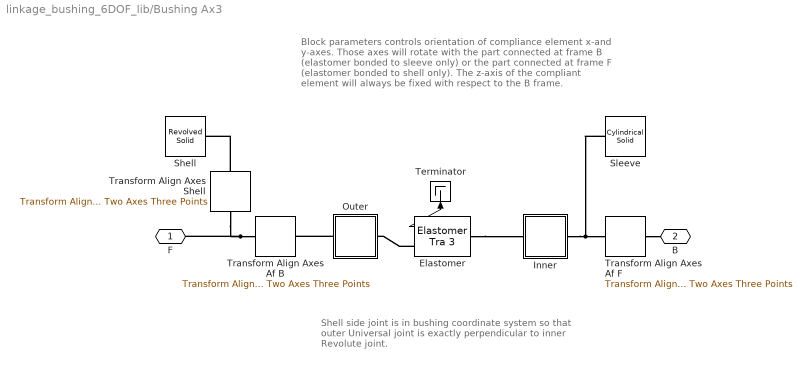
== system linkage_bushing_6DOF_lib/Bushing Ax3 ==
  note: Shell side joint is in bushing coordinate system so that outer Universal joint is exactly perpendicular to inner Revolute joint.
  note: Block parameters controls orientation of compliance element x-and y-axes. Those axes will rotate with the part connected at frame B (elastomer bonded to sleeve only) or the part connected at frame F (elastomer bonded to shell only). The z-axis of the compliant element will always be fixed with respect to the B frame.
  Elastomer : linkage_bushing_5DOF_lib/Elastomer Tra 3  checkbox_setTargets=on  popup_force_law_spr_axiX=Linear  k_axialX=sprx.Linear.K.Value  x_axialX=sprx.Table.x.Value  f_axialX_spr=sprx.Table.f.Value  popup_force_law_dam_axiX=Linear  d_axialX=damx.Linear.d.Value  v_axialX=damx.Table.v.Value  f_axialX_dam=damx.Table.f.Value  popup_force_law_spr_axiY=Linear  k_axialY=spry.Linear.K.Value  x_axialY=spry.Table.x.Value  f_axialY_spr=spry.Table.f.Value  popup_force_law_dam_axiY=Linear  d_axialY=damy.Linear.d.Value  v_axialY=damy.Table.v.Value  f_axialY_dam=damy.Table.f.Value  popup_force_law_spr_axiZ=Linear  k_axialZ=sprz.Linear.K.Value  x_axialZ=sprz.Table.x.Value  f_axialZ_spr=sprz.Table.f.Value  popup_force_law_dam_axiZ=Linear  d_axialZ=damz.Linear.d.Value  v_axialZ=damz.Table.v.Value  f_axialZ_dam=damz.Table.f.Value  shell_or=shell_or  elastomer_ir=Visual.hp.rad  shell_len=shell_len  elastomer_clr=Visual.Bushing.clr  elastomer_opc=Visual.part.opc  elastomer_axis_clr=Visual.BushingXAxis.clr
  Inner : Subsystem  Variant=on  VariantControlMode=label  VariantControl=Choice  LabelModeActiveChoice=Revolute  mask{checkbox_setTargets=on}
      mask prompts: checkbox_setTargets "Set position targets to 0"
      mask init:
      | curblk = gcb;
      | set_param([curblk '/Revolute'],'checkbox_setTargets',checkbox_setTargets)
      settings: AttributesFormatString=%<LabelModeActiveChoice>
  Outer : Subsystem  Variant=on  VariantControlMode=label  VariantControl=Choice  LabelModeActiveChoice=Universal  mask{checkbox_setTargets=on}
      mask prompts: checkbox_setTargets "Set position targets to 0"
      mask init:
      | curblk = gcb;
      | set_param([curblk '/Universal'],'checkbox_setTargets',checkbox_setTargets);
      | set_param([curblk '/Gimbal'],'checkbox_setTargets',checkbox_setTargets);
      settings: AttributesFormatString=%<LabelModeActiveChoice>
  Shell : sm_lib/Body Elements/Revolved Solid  RevolutionCrossSection=[shell_or*0.95 0.5; shell_or*0.95 -0.5; shell_or -0.5; shell_or 0.5].*[1 shell_len]  RevolutionCrossSectionUnits=m  RevolutionExtent=Full  RevolutionAngle=180  RevolutionAngleUnits=deg  ExportConvexHullGeometry=off  InertiaType=CalculateFromGeometry  BasedOnType=Density  Density=1  DensityUnits=kg/m^3  Mass=1  MassUnits=kg  CenterOfMass=[0 0 0]  CenterOfMassUnits=m  MomentsOfInertia=[1 1 1]  MomentsOfInertiaUnits=kg*m^2  ProductsOfInertia=[0 0 0]  ProductsOfInertiaUnits=kg*m^2  GraphicType=FromGeometry  MarkerShape=Sphere  MarkerSize=10  GraphicVisPropType=SimpleVisualProperties  GraphicDiffuseColor=shell_clr  GraphicOpacity=shell_opc  GraphicSpecularColor=[0.5 0.5 0.5 1.0]  GraphicAmbientColor=[0.15 0.15 0.15 1.0]  GraphicEmissiveColor=[0.0 0.0 0.0 1.0]  GraphicShininess=75  DoExposeReferenceFrame=on  SerializedFrames=<Frames/>
  Sleeve : sm_lib/Body Elements/Cylindrical Solid  CylinderRadius=shell_or/4  CylinderRadiusUnits=m  CylinderLength=shell_len  CylinderLengthUnits=m  ExportEntireGeometry=off  InertiaType=CalculateFromGeometry  BasedOnType=Density  Density=1  DensityUnits=kg/m^3  Mass=1  MassUnits=kg  CenterOfMass=[0 0 0]  CenterOfMassUnits=m  MomentsOfInertia=[1 1 1]  MomentsOfInertiaUnits=kg*m^2  ProductsOfInertia=[0 0 0]  ProductsOfInertiaUnits=kg*m^2  GraphicType=FromGeometry  MarkerShape=Sphere  MarkerSize=10  GraphicVisPropType=SimpleVisualProperties  GraphicDiffuseColor=sleeve_clr  GraphicOpacity=sleeve_opc  GraphicSpecularColor=[0.5 0.5 0.5 1.0]  GraphicAmbientColor=[0.15 0.15 0.15 1.0]  GraphicEmissiveColor=[0.0 0.0 0.0 1.0]  GraphicShininess=75  DoExposeReferenceFrame=on  SerializedFrames=<Frames/>
  Terminator : Terminator
  Transform Align Axes Af B : Suspension_Utilities/Transform Align Two Axes Three Points  hpo=hp_j.*leftOrRight_vec  hpz=hp_z.*leftOrRight_vec  hpx=hp_x.*leftOrRight_vec
  Transform Align Axes Af F : Suspension_Utilities/Transform Align Two Axes Three Points  hpo=hp_j.*leftOrRight_vec  hpz=hp_z.*leftOrRight_vec  hpx=hp_x.*leftOrRight_vec
  Transform Align Axes Shell : Suspension_Utilities/Transform Align Two Axes Three Points  hpo=hp_j.*leftOrRight_vec  hpz=hp_z.*leftOrRight_vec  hpx=hp_x.*leftOrRight_vec
  F : PMIOPort  Side=Right
  " B" : PMIOPort  Port=2  Side=Left
  wires:
  Elastomer/1 -> Terminator/1
  connections:
  Outer/LConn1 -- Transform Align Axes Af B/RConn1
  Transform Align Axes Af F/LConn1 -- " B"/RConn1
  Inner/LConn1 -- Sleeve/RConn1 -- Transform Align Axes Af F/RConn1
  Elastomer/LConn1 -- Inner/RConn1
  Transform Align Axes Af B/LConn1 -- F/RConn1 -- Transform Align Axes Shell/LConn1
  Transform Align Axes Shell/RConn1 -- Shell/RConn1
  Elastomer/RConn1 -- Outer/RConn1

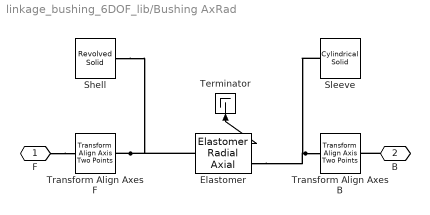
== system linkage_bushing_6DOF_lib/Bushing AxRad ==
  Elastomer : $bdroot/Elastomer Radial Axial  checkbox_setTargets=on  popup_force_law_spr_rad=Linear  k_radial=sprRad.Linear.K.Value  x_radial=sprRad.Table.x.Value  f_radial_spr=sprRad.Table.f.Value  k1_radial_max=sprRad.Maxwell.k1.Value  b1_radial_max=sprRad.Maxwell.b1.Value  x_radial_max=sprRad.Maxwell.x.Value  f_radial_max=sprRad.Maxwell.f.Value  popup_force_law_dam_rad=Linear  d_radial=damRad.Linear.d.Value  v_radial=damRad.Table.v.Value  f_radial_dam=damRad.Table.f.Value  popup_force_law_spr_axi=Linear  k_axial=sprAxi.Linear.K.Value  x_axial=sprAxi.Table.x.Value  f_axial_spr=sprAxi.Table.f.Value  popup_force_law_dam_axi=Linear  d_axial=damAxi.Linear.d.Value  v_axial=damAxi.Linear.v.Value  f_axial_dam=damAxi.Linear.f.Value  shell_or=Visual.hp.rad*2  elastomer_ir=Visual.hp.rad  shell_len=Visual.hp.rad*2  elastomer_clr=Visual.Bushing.clr  elastomer_opc=Visual.part.opc
  Shell : sm_lib/Body Elements/Revolved Solid  RevolutionCrossSection=[shell_or*0.95 0.5; shell_or*0.95 -0.5; shell_or -0.5; shell_or 0.5].*[1 shell_len]  RevolutionCrossSectionUnits=m  RevolutionExtent=Full  RevolutionAngle=180  RevolutionAngleUnits=deg  ExportConvexHullGeometry=off  InertiaType=CalculateFromGeometry  BasedOnType=Density  Density=1  DensityUnits=kg/m^3  Mass=1  MassUnits=kg  CenterOfMass=[0 0 0]  CenterOfMassUnits=m  MomentsOfInertia=[1 1 1]  MomentsOfInertiaUnits=kg*m^2  ProductsOfInertia=[0 0 0]  ProductsOfInertiaUnits=kg*m^2  GraphicType=FromGeometry  MarkerShape=Sphere  MarkerSize=10  GraphicVisPropType=SimpleVisualProperties  GraphicDiffuseColor=shell_clr  GraphicOpacity=shell_opc  GraphicSpecularColor=[0.5 0.5 0.5 1.0]  GraphicAmbientColor=[0.15 0.15 0.15 1.0]  GraphicEmissiveColor=[0.0 0.0 0.0 1.0]  GraphicShininess=75  DoExposeReferenceFrame=on  SerializedFrames=<Frames/>
  Sleeve : sm_lib/Body Elements/Cylindrical Solid  CylinderRadius=shell_or/4  CylinderRadiusUnits=m  CylinderLength=shell_len  CylinderLengthUnits=m  ExportEntireGeometry=off  InertiaType=CalculateFromGeometry  BasedOnType=Density  Density=1  DensityUnits=kg/m^3  Mass=1  MassUnits=kg  CenterOfMass=[0 0 0]  CenterOfMassUnits=m  MomentsOfInertia=[1 1 1]  MomentsOfInertiaUnits=kg*m^2  ProductsOfInertia=[0 0 0]  ProductsOfInertiaUnits=kg*m^2  GraphicType=FromGeometry  MarkerShape=Sphere  MarkerSize=10  GraphicVisPropType=SimpleVisualProperties  GraphicDiffuseColor=sleeve_clr  GraphicOpacity=sleeve_opc  GraphicSpecularColor=[0.5 0.5 0.5 1.0]  GraphicAmbientColor=[0.15 0.15 0.15 1.0]  GraphicEmissiveColor=[0.0 0.0 0.0 1.0]  GraphicShininess=75  DoExposeReferenceFrame=on  SerializedFrames=<Frames/>
  Terminator : Terminator
  Transform Align Axes B : Suspension_Utilities/Transform Align Axis Two Points  hp_b=hp_j.*leftOrRight_vec  hp_t=hp_z.*leftOrRight_vec  popup_f_axis=+Z
  Transform Align Axes F : Suspension_Utilities/Transform Align Axis Two Points  hp_b=hp_j.*leftOrRight_vec  hp_t=hp_z.*leftOrRight_vec  popup_f_axis=+Z
  F : PMIOPort  Side=Right
  " B" : PMIOPort  Port=2  Side=Left
  wires:
  Elastomer/1 -> Terminator/1
  connections:
  Transform Align Axes F/RConn1 -- Elastomer/LConn1 -- Shell/RConn1
  Transform Align Axes B/RConn1 -- Elastomer/RConn1 -- Sleeve/RConn1
  " B"/RConn1 -- Transform Align Axes B/LConn1
  F/RConn1 -- Transform Align Axes F/LConn1
